simulink model "tb_rc_link"  (R2026b)
values from neighbouring files (symbols this model uses):
  Ts = prm.Ts    [row_driver_bench.m]
settings Model: Creator=aomar  LastModifiedBy=aomar

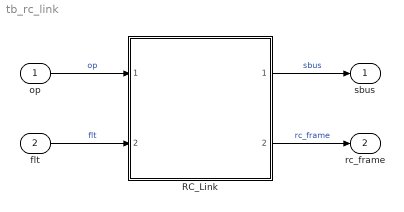
== system tb_rc_link ==
  op : Inport  OutDataTypeStr=Bus: Bus_OperatorCmd  SampleTime=Ts.ctrl  BusOutputAsStruct=on
  flt : Inport  Port=2  OutDataTypeStr=Bus: Bus_FaultInject  SampleTime=Ts.ctrl  BusOutputAsStruct=on
  RC_Link : Subsystem  ReferencedSubsystem=RC_Link_Sim
  sbus : Outport  OutDataTypeStr=Bus: Bus_SbusStream
  rc_frame : Outport  Port=2  OutDataTypeStr=Bus: Bus_RcFrame
  wires:
  op/1 -> RC_Link/1  "op"
  flt/1 -> RC_Link/2  "flt"
  RC_Link/1 -> sbus/1  "sbus"
  RC_Link/2 -> rc_frame/1  "rc_frame"
